simulink model "untitled2"  (R2026b)
settings: Solver=VariableStepAuto  StopTime=5.0  MaxStep=1e-3
values from neighbouring files (symbols this model uses):
  comdelay = 0.02    [parametro2.m]
  pninv = 2000    [parametro2.m]
  tau_pv = 0.5    [parametro2.m]
  tsample = 0.2    [parametro2.m]
libraries: sl_discontinuities x5
settings Model: Creator=paulo.delgado  LastModifiedBy=ArnauCoronado

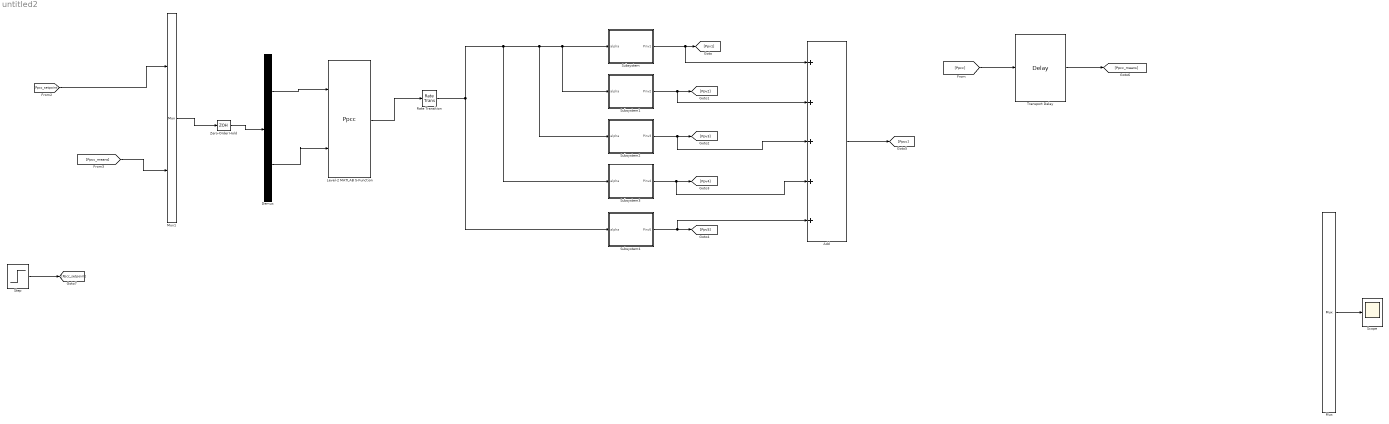
== system untitled2 ==
  Add : Sum  Inputs=+++++
  Demux : Demux  Outputs=2
  Level-2 MATLAB S-Function : M-S-Function  FunctionName=Ppcc
  Mux : Mux  Inputs=5
  Mux1 : Mux  Inputs=2
  Rate Transition : RateTransition
  Scope : Scope
      settings: ActiveDisplayYMinimum=-249.99999999999994  ActiveDisplayYMaximum=2250
  Step : Step  Time=0.5  InitialValue=10000  FinalValue=0  SampleTime=0
  Subsystem : Subsystem
  Subsystem1 : Subsystem
  Subsystem2 : Subsystem
  Subsystem3 : Subsystem
  Subsystem4 : Subsystem
  Transport Delay : TransportDelay  DelayTime=comdelay
  Zero-Order Hold : ZeroOrderHold  SampleTime=tsample
  wires:
  Mux/1 -> Scope/1
  Subsystem/1(Pinv1) -> Add/1, [Ppv1]
  Subsystem1/1(Pinv2) -> Add/2, [Ppv2]
  Subsystem2/1(Pinv3) -> Add/3, [Ppv3]
  Subsystem3/1(Pinv4) -> Add/4, [Ppv4]
  Subsystem4/1(Pinv5) -> Add/5, [Ppv5]
  Rate Transition/1 -> Subsystem3/1(alpha), Subsystem2/1(alpha), Subsystem1/1(alpha), Subsystem/1(alpha), Subsystem4/1(alpha)
  Add/1 -> [Ppcc]
  [Ppcc] -> Transport Delay/1
  Transport Delay/1 -> [Ppcc_means]
  Step/1 -> [Ppcc_setpoint]
  Mux1/1 -> Zero-Order Hold/1
  [Ppcc_setpoint] -> Mux1/1
  [Ppcc_means] -> Mux1/2
  Zero-Order Hold/1 -> Demux/1
  Demux/1 -> Level-2 MATLAB S-Function/1
  Demux/2 -> Level-2 MATLAB S-Function/2
  Level-2 MATLAB S-Function/1 -> Rate Transition/1

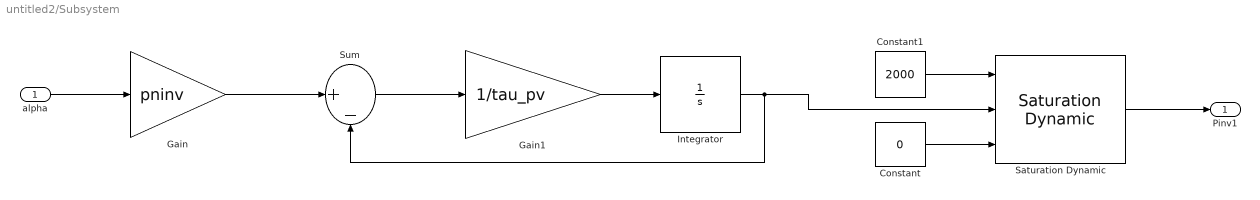
== system untitled2/Subsystem ==
  alpha : Inport
  Constant : Constant  Value=0
  Constant1 : Constant  Value=2000
  Gain : Gain  Gain=pninv
  Gain1 : Gain  Gain=1/tau_pv
  Integrator : Integrator  InitialCondition=2000
  Saturation Dynamic : sl_discontinuities/Saturation Dynamic  OutMin=[]  OutMax=[]  OutDataTypeStr=Inherit: Same as second input  OutDataType=fixdt(1, 16)  OutScaling=2^-10  DoSatur=off
      settings: LibrarySourceBlock=|
      | simulink/Discontinuities/Saturation
      | Dynamic
  Sum : Sum  Inputs=|+-
  Pinv1 : Outport
  wires:
  Integrator/1 -> Saturation Dynamic/2, Sum/2
  Constant/1 -> Saturation Dynamic/3
  Sum/1 -> Gain1/1
  Gain1/1 -> Integrator/1
  Saturation Dynamic/1 -> Pinv1/1
  Gain/1 -> Sum/1
  Constant1/1 -> Saturation Dynamic/1
  alpha/1 -> Gain/1

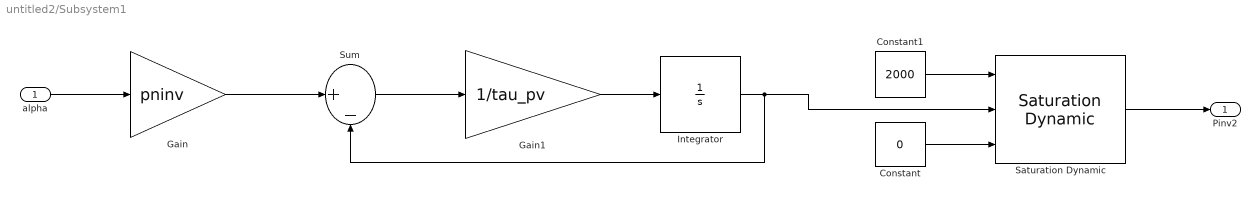
== system untitled2/Subsystem1 ==
  alpha : Inport
  Constant : Constant  Value=0
  Constant1 : Constant  Value=2000
  Gain : Gain  Gain=pninv
  Gain1 : Gain  Gain=1/tau_pv
  Integrator : Integrator  InitialCondition=2000
  Saturation Dynamic : sl_discontinuities/Saturation Dynamic  OutMin=[]  OutMax=[]  OutDataTypeStr=Inherit: Same as second input  OutDataType=fixdt(1, 16)  OutScaling=2^-10  DoSatur=off
      settings: LibrarySourceBlock=|
      | simulink/Discontinuities/Saturation
      | Dynamic
  Sum : Sum  Inputs=|+-
  Pinv2 : Outport
  wires:
  alpha/1 -> Gain/1
  Constant1/1 -> Saturation Dynamic/1
  Gain/1 -> Sum/1
  Saturation Dynamic/1 -> Pinv2/1
  Gain1/1 -> Integrator/1
  Sum/1 -> Gain1/1
  Constant/1 -> Saturation Dynamic/3
  Integrator/1 -> Sum/2, Saturation Dynamic/2

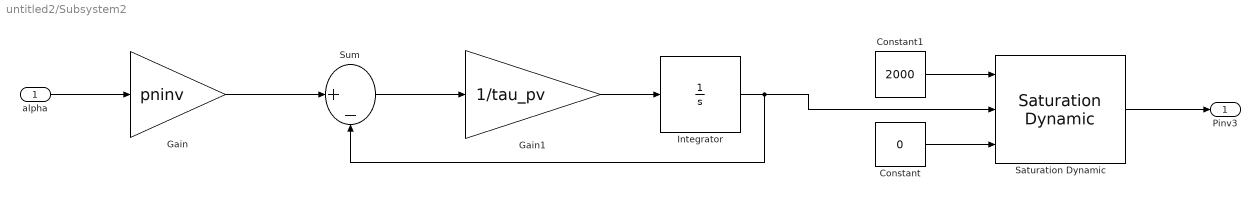
== system untitled2/Subsystem2 ==
  alpha : Inport
  Constant : Constant  Value=0
  Constant1 : Constant  Value=2000
  Gain : Gain  Gain=pninv
  Gain1 : Gain  Gain=1/tau_pv
  Integrator : Integrator  InitialCondition=2000
  Saturation Dynamic : sl_discontinuities/Saturation Dynamic  OutMin=[]  OutMax=[]  OutDataTypeStr=Inherit: Same as second input  OutDataType=fixdt(1, 16)  OutScaling=2^-10  DoSatur=off
      settings: LibrarySourceBlock=|
      | simulink/Discontinuities/Saturation
      | Dynamic
  Sum : Sum  Inputs=|+-
  Pinv3 : Outport
  wires:
  Integrator/1 -> Saturation Dynamic/2, Sum/2
  Constant/1 -> Saturation Dynamic/3
  Sum/1 -> Gain1/1
  Gain1/1 -> Integrator/1
  Saturation Dynamic/1 -> Pinv3/1
  Gain/1 -> Sum/1
  Constant1/1 -> Saturation Dynamic/1
  alpha/1 -> Gain/1

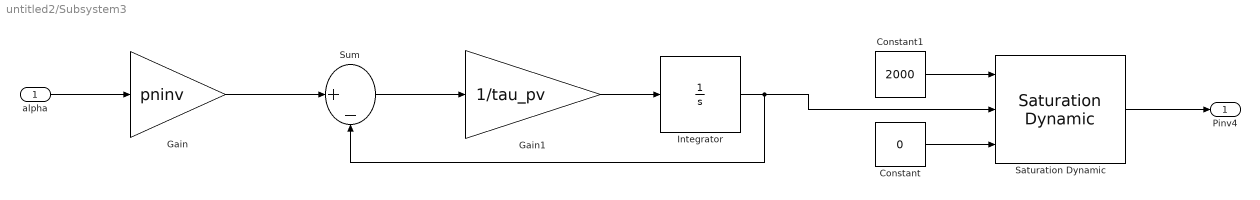
== system untitled2/Subsystem3 ==
  alpha : Inport
  Constant : Constant  Value=0
  Constant1 : Constant  Value=2000
  Gain : Gain  Gain=pninv
  Gain1 : Gain  Gain=1/tau_pv
  Integrator : Integrator  InitialCondition=2000
  Saturation Dynamic : sl_discontinuities/Saturation Dynamic  OutMin=[]  OutMax=[]  OutDataTypeStr=Inherit: Same as second input  OutDataType=fixdt(1, 16)  OutScaling=2^-10  DoSatur=off
      settings: LibrarySourceBlock=|
      | simulink/Discontinuities/Saturation
      | Dynamic
  Sum : Sum  Inputs=|+-
  Pinv4 : Outport
  wires:
  alpha/1 -> Gain/1
  Constant1/1 -> Saturation Dynamic/1
  Gain/1 -> Sum/1
  Saturation Dynamic/1 -> Pinv4/1
  Gain1/1 -> Integrator/1
  Sum/1 -> Gain1/1
  Constant/1 -> Saturation Dynamic/3
  Integrator/1 -> Sum/2, Saturation Dynamic/2

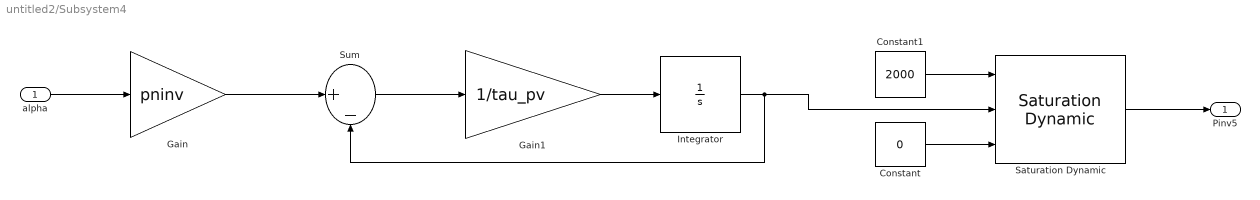
== system untitled2/Subsystem4 ==
  alpha : Inport
  Constant : Constant  Value=0
  Constant1 : Constant  Value=2000
  Gain : Gain  Gain=pninv
  Gain1 : Gain  Gain=1/tau_pv
  Integrator : Integrator  InitialCondition=2000
  Saturation Dynamic : sl_discontinuities/Saturation Dynamic  OutMin=[]  OutMax=[]  OutDataTypeStr=Inherit: Same as second input  OutDataType=fixdt(1, 16)  OutScaling=2^-10  DoSatur=off
      settings: LibrarySourceBlock=|
      | simulink/Discontinuities/Saturation
      | Dynamic
  Sum : Sum  Inputs=|+-
  Pinv5 : Outport
  wires:
  Integrator/1 -> Saturation Dynamic/2, Sum/2
  Constant/1 -> Saturation Dynamic/3
  Sum/1 -> Gain1/1
  Gain1/1 -> Integrator/1
  Saturation Dynamic/1 -> Pinv5/1
  Gain/1 -> Sum/1
  Constant1/1 -> Saturation Dynamic/1
  alpha/1 -> Gain/1
